simulink model "DCHR_Dispatch_Stateflow_v28"  (R2026a)
settings: Solver=FixedStepDiscrete  StopTime=dchr_stop_v28  FixedStep=dchr_dt_v28
model workspace (MAT data in the model file):
  dchr_E0_v28 = 0
  dchr_dt_v28 = 1
  dchr_h_v28 = [8 0.45 1.2 8 0.08 0 4 0 0]
  dchr_input_v28 = [0  6  35  70  5; 1  0  35  70  6; 2  0  35  70  10]
  dchr_p_v28 = [1 10 3 4 0.9 0.8 0.01 2]
  dchr_stop_v28 = 2
settings Model: Creator=Lysda  LastModifiedBy=Lysda

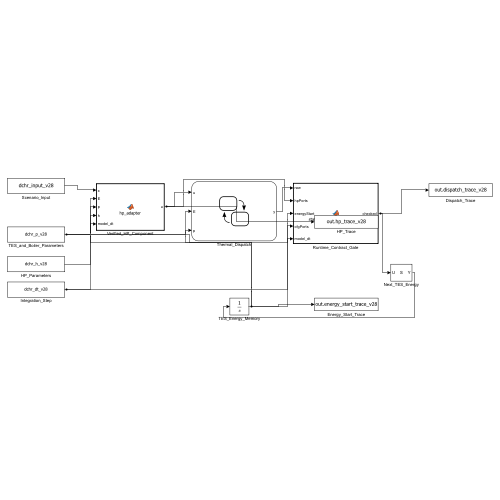
[thumbnail: Simulink's stored preview of the top-level diagram]
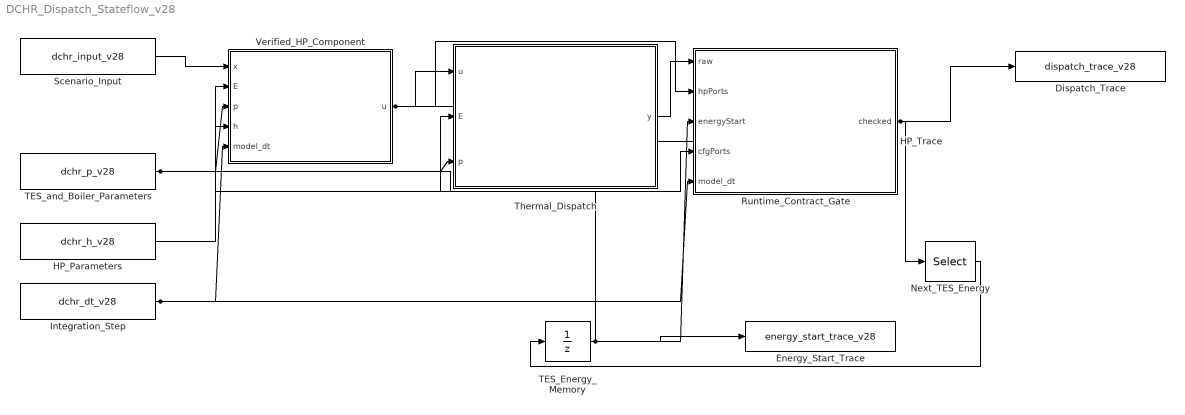
== system DCHR_Dispatch_Stateflow_v28 ==
  Dispatch_Trace : ToWorkspace  VariableName=dispatch_trace_v28  SaveFormat=Timeseries  SampleTime=-1
  Energy_Start_Trace : ToWorkspace  VariableName=energy_start_trace_v28  SaveFormat=Timeseries  SampleTime=-1
  HP_Parameters : Constant  Value=dchr_h_v28
  HP_Trace : ToWorkspace  VariableName=hp_trace_v28  SaveFormat=Timeseries  SampleTime=-1
  Integration_Step : Constant  Value=dchr_dt_v28
  Next_TES_Energy : Selector  InputPortWidth=13  IndexOptions=Index vector (dialog)  Indices=8  OutputSizes=1
  Runtime_Contract_Gate : MATLAB Function  TreatAsAtomicUnit=on
  Scenario_Input : FromWorkspace  VariableName=dchr_input_v28  SampleTime=dchr_dt_v28  Interpolate=off  OutputAfterFinalValue=Holding final value
  TES_Energy_Memory : UnitDelay  InitialCondition=dchr_E0_v28  SampleTime=dchr_dt_v28
  TES_and_Boiler_Parameters : Constant  Value=dchr_p_v28
  Thermal_Dispatch : Stateflow chart  TreatAsAtomicUnit=on
  Verified_HP_Component : MATLAB Function  TreatAsAtomicUnit=on
  wires:
  Scenario_Input/1 -> Verified_HP_Component/1(x)
  TES_Energy_Memory/1 -> Verified_HP_Component/2(E), Thermal_Dispatch/2(E), Runtime_Contract_Gate/3(energyStart), Energy_Start_Trace/1
  TES_and_Boiler_Parameters/1 -> Verified_HP_Component/3(p), Thermal_Dispatch/3(p), Runtime_Contract_Gate/4(cfgPorts)
  HP_Parameters/1 -> Verified_HP_Component/4(h)
  Verified_HP_Component/1(u) -> Thermal_Dispatch/1(u), Runtime_Contract_Gate/2(hpPorts), HP_Trace/1
  Integration_Step/1 -> Verified_HP_Component/5(model_dt), Runtime_Contract_Gate/5(model_dt)
  Thermal_Dispatch/1(y) -> Runtime_Contract_Gate/1(raw)
  Runtime_Contract_Gate/1(checked) -> Next_TES_Energy/1, Dispatch_Trace/1
  Next_TES_Energy/1 -> TES_Energy_Memory/1

== matlab function DCHR_Dispatch_Stateflow_v28/Runtime_Contract_Gate ==
  data: raw input; checked output; hpPorts input; energyStart input; cfgPorts input; model_dt input
function checked = stateflow_contract_gate_v28(raw,hpPorts,energyStart,cfgPorts,model_dt)
%#codegen
% Executed after the operational chart, before accepted trace/TES feedback.
% Powers MW; energies MWh; dt h. Exponential passive retention, LOSS-FIRST split.
% Constant ambient/property lumped assumption; active-flow integration is approximate.
dt=cfgPorts(1); cap=cfgPorts(2); etaC=cfgPorts(5); etaD=cfgPorts(6);
assert(isfinite(model_dt) && model_dt>0 && dt==model_dt, ...
    'Physical interval must equal the model sample time.');
assert(cfgPorts(7)>=0 && isfinite(cfgPorts(7)*dt), 'Invalid continuous loss-rate product.');
assert(all(isfinite(raw)) && all(isfinite(cfgPorts)), ...
    'Accepted dispatch and parameters must be finite.');
assert(all(isfinite(hpPorts([1 2 3 4 5 7 8]))), ...
    'HP ports except off-state COP must be finite.');
% Scale tolerance with total interval energy, never with a reported residual.
scale=max(1,abs(energyStart)+(abs(hpPorts(2))+abs(cfgPorts(8)))*dt+abs(cap));
tol=1e-10*scale;
powerTol=tol/max(dt,eps);
assert(isfinite(scale) && isfinite(tol) && isfinite(powerTol), 'Overflow in contract tolerance.');
assert(energyStart>=0 && energyStart<=cap && cap>=0, 'TES start outside capacity.');
assert(all(raw([2:6 12])>=-powerTol) && all(raw(7:11)>=-tol) && ...
    all(hpPorts([1 2 3 4 5 7 8])>=0), ...
    'Negative dispatch/HP port.');
assert(raw(1)==floor(raw(1)) && raw(1)>=0 && raw(1)<=5, 'Undefined mode.');
assert(raw(3)<=cfgPorts(3)+powerTol && raw(4)<=cfgPorts(4)+powerTol && ...
    raw(5)<=cfgPorts(8)+powerTol, 'TES/backup power limit exceeded.');
assert(raw(7)>=-tol && raw(7)<=cap+tol && raw(8)>=-tol && raw(8)<=cap+tol, ...
    'TES state outside capacity.');
assert(raw(3)*raw(4)==0, 'Simultaneous TES charge and discharge.');
assert(abs(hpPorts(2)-hpPorts(3)-hpPorts(4))*dt<=tol, 'HP first-law failure.');
assert(abs(hpPorts(2)-raw(2)-raw(3))*dt<=tol, 'Unallocated HP condenser heat.');
assert(abs(hpPorts(1)-raw(2)-raw(4)-raw(5)-raw(6))*dt<=tol, 'Demand closure failure.');
assert(abs(raw(12)-raw(2)-raw(4)-raw(5))*dt<=tol, 'Useful heat mismatch.');
assert(abs(raw(7)-energyStart*exp(-cfgPorts(7)*dt))<=tol, 'Standing-retention mismatch.');
assert(abs(raw(9)-(energyStart-raw(7)))<=tol && ...
    abs(raw(10)-(1-etaC)*raw(3)*dt)<=tol && ...
    abs(raw(11)-(1/etaD-1)*raw(4)*dt)<=tol, 'TES loss reporting mismatch.');
tesResidual=energyStart+(raw(3)-raw(4))*dt-raw(8)-sum(raw(9:11));
assert(abs(tesResidual)<=tol, 'TES first-law failure.');
systemResidual=(hpPorts(4)+hpPorts(3)+raw(5))*dt+energyStart ...
    -raw(12)*dt-raw(8)-sum(raw(9:11));
assert(abs(systemResidual)<=tol && abs(raw(13)-systemResidual)<=tol, ...
    'System first-law failure or false residual.');
expected=0;
if raw(6)>0, expected=5;
elseif raw(5)>0, expected=4;
elseif raw(4)>0, expected=3;
elseif raw(3)>0, expected=2;
elseif raw(2)>0, expected=1;
end
assert(raw(1)==expected, 'Active state does not match delivered flows.');
if hpPorts(2)>0
    assert(isfinite(hpPorts(6)) && hpPorts(6)>1 && hpPorts(7)==1, 'Invalid operating COP/availability.');
    assert(abs(hpPorts(3)*hpPorts(6)-hpPorts(2))*dt<=tol, 'COP port inconsistency.');
else
    assert(isnan(hpPorts(6)) && hpPorts(7)==0, 'Off HP must have undefined COP.');
end
checked=raw;
end

== matlab function DCHR_Dispatch_Stateflow_v28/Verified_HP_Component ==
  data: x input; u output; E input; p input; h input; model_dt input
function u=hp_adapter(x,E,p,h,model_dt)
%#codegen
coder.extrinsic('dchr_stateflow_hp_v28');
u=zeros(8,1);
u=dchr_stateflow_hp_v28(x,E,p,h,model_dt);
end

== stateflow chart DCHR_Dispatch_Stateflow_v28/Thermal_Dispatch ==
  settings: updateMethod=DISCRETE  sampleTime=dchr_dt_v28  description=v28 exponential passive TES retention; loss-first split. Six-state finite TES/HP/boiler dispatch. Normal-mode host HP component; state actions drive all delivery ports.
  state IDLE
    en,du:
    y=stateflow_allocate_v28(0,u,E,p);
  state HEAT_RECOVERY
    en,du:
    y=stateflow_allocate_v28(1,u,E,p);
  state STORAGE_CHARGE
    en,du:
    y=stateflow_allocate_v28(2,u,E,p);
  state STORAGE_DISCHARGE
    en,du:
    y=stateflow_allocate_v28(3,u,E,p);
  state BACKUP
    en,du:
    y=stateflow_allocate_v28(4,u,E,p);
  state UNMET_DEMAND
    en,du:
    y=stateflow_allocate_v28(5,u,E,p);
  (junction 22) -> STORAGE_CHARGE [order 3] : [stateflow_choose_mode_v28(u,E,p)==2]
  (junction 22) -> HEAT_RECOVERY [order 2] : [stateflow_choose_mode_v28(u,E,p)==1]
  (default) -> (junction 22)
  (junction 22) -> IDLE [order 1] : [stateflow_choose_mode_v28(u,E,p)==0]
  (junction 22) -> UNMET_DEMAND [order 6] : [stateflow_choose_mode_v28(u,E,p)==5]
  (junction 22) -> STORAGE_DISCHARGE [order 4] : [stateflow_choose_mode_v28(u,E,p)==3]
  (junction 22) -> BACKUP [order 5] : [stateflow_choose_mode_v28(u,E,p)==4]
  STORAGE_CHARGE -> STORAGE_DISCHARGE [order 3] : [stateflow_choose_mode_v28(u,E,p)==3]
  HEAT_RECOVERY -> STORAGE_DISCHARGE [order 3] : [stateflow_choose_mode_v28(u,E,p)==3]
  STORAGE_CHARGE -> BACKUP [order 4] : [stateflow_choose_mode_v28(u,E,p)==4]
  STORAGE_DISCHARGE -> IDLE [order 1] : [stateflow_choose_mode_v28(u,E,p)==0]
  UNMET_DEMAND -> IDLE [order 1] : [stateflow_choose_mode_v28(u,E,p)==0]
  STORAGE_CHARGE -> IDLE [order 1] : [stateflow_choose_mode_v28(u,E,p)==0]
  BACKUP -> IDLE [order 1] : [stateflow_choose_mode_v28(u,E,p)==0]
  HEAT_RECOVERY -> IDLE [order 1] : [stateflow_choose_mode_v28(u,E,p)==0]
  STORAGE_DISCHARGE -> HEAT_RECOVERY [order 2] : [stateflow_choose_mode_v28(u,E,p)==1]
  STORAGE_DISCHARGE -> STORAGE_CHARGE [order 3] : [stateflow_choose_mode_v28(u,E,p)==2]
  BACKUP -> HEAT_RECOVERY [order 2] : [stateflow_choose_mode_v28(u,E,p)==1]
  IDLE -> HEAT_RECOVERY [order 1] : [stateflow_choose_mode_v28(u,E,p)==1]
  IDLE -> STORAGE_CHARGE [order 2] : [stateflow_choose_mode_v28(u,E,p)==2]
  UNMET_DEMAND -> HEAT_RECOVERY [order 2] : [stateflow_choose_mode_v28(u,E,p)==1]
  STORAGE_CHARGE -> HEAT_RECOVERY [order 2] : [stateflow_choose_mode_v28(u,E,p)==1]
  BACKUP -> STORAGE_CHARGE [order 3] : [stateflow_choose_mode_v28(u,E,p)==2]
  UNMET_DEMAND -> STORAGE_CHARGE [order 3] : [stateflow_choose_mode_v28(u,E,p)==2]
  HEAT_RECOVERY -> STORAGE_CHARGE [order 2] : [stateflow_choose_mode_v28(u,E,p)==2]
  IDLE -> STORAGE_DISCHARGE [order 3] : [stateflow_choose_mode_v28(u,E,p)==3]
  HEAT_RECOVERY -> BACKUP [order 4] : [stateflow_choose_mode_v28(u,E,p)==4]
  STORAGE_CHARGE -> UNMET_DEMAND [order 5] : [stateflow_choose_mode_v28(u,E,p)==5]
  IDLE -> BACKUP [order 4] : [stateflow_choose_mode_v28(u,E,p)==4]
  IDLE -> UNMET_DEMAND [order 5] : [stateflow_choose_mode_v28(u,E,p)==5]
  HEAT_RECOVERY -> UNMET_DEMAND [order 5] : [stateflow_choose_mode_v28(u,E,p)==5]
  UNMET_DEMAND -> STORAGE_DISCHARGE [order 4] : [stateflow_choose_mode_v28(u,E,p)==3]
  BACKUP -> STORAGE_DISCHARGE [order 4] : [stateflow_choose_mode_v28(u,E,p)==3]
  STORAGE_DISCHARGE -> BACKUP [order 4] : [stateflow_choose_mode_v28(u,E,p)==4]
  STORAGE_DISCHARGE -> UNMET_DEMAND [order 5] : [stateflow_choose_mode_v28(u,E,p)==5]
  UNMET_DEMAND -> BACKUP [order 5] : [stateflow_choose_mode_v28(u,E,p)==4]
  BACKUP -> UNMET_DEMAND [order 5] : [stateflow_choose_mode_v28(u,E,p)==5]
  data: hpPorts function_input; energyStart function_input; cfgPorts function_input; mode function_output; mode function_input; hpPorts function_input; energyStart function_input; cfgPorts function_input; y function_output; u input double size=[8 1]; E input double size=1; p input double size=[1 8]; y output double size=[13 1]
  function mode = stateflow_choose_mode_v28(hpPorts,energyStart,cfgPorts):
    | function mode = stateflow_choose_mode_v28(hpPorts,energyStart,cfgPorts)
    | %#codegen
    | % Highest service condition; BACKUP/UNMET can include HP and TES discharge.
    | % hpPorts = [demand, HP heat, electricity, source used, request, COP, available, unused]
    | % cfgPorts = [dt_h, capacity, charge limit, discharge limit, etaC, etaD, continuous lambda/h, boiler]
    | after=energyStart*exp(-cfgPorts(7)*cfgPorts(1));
    | direct=min(hpPorts(1),hpPorts(2));
    | discharge=min([max(0,hpPorts(1)-direct),cfgPorts(4),after*cfgPorts(6)/cfgPorts(1)]);
    | remaining=max(0,hpPorts(1)-direct-discharge);
    | if remaining>cfgPorts(8)
    |     mode=5;
    | elseif remaining>0
    |     mode=4;
    | elseif discharge>0
    |     mode=3;
    | elseif hpPorts(2)>direct
    |     mode=2;
    | elseif direct>0
    |     mode=1;
    | else
    |     mode=0;
    | end
    | end
  function y = stateflow_allocate_v28(mode,hpPorts,energyStart,cfgPorts):
    | function y = stateflow_allocate_v28(mode,hpPorts,energyStart,cfgPorts)
    | %#codegen
    | % Called by the active Stateflow state's entry and during actions.
    | % States determine which TES/backup/unmet ports may operate.
    | dt=cfgPorts(1); after=energyStart*exp(-cfgPorts(7)*dt);
    | direct=0; charge=0; discharge=0; gas=0; unmet=0;
    | if mode>=1
    |     direct=min(hpPorts(1),hpPorts(2));
    | end
    | if mode==2
    |     charge=min([max(0,hpPorts(2)-direct),cfgPorts(3),(cfgPorts(2)-after)/dt/cfgPorts(5)]);
    | end
    | if mode>=3
    |     discharge=min([max(0,hpPorts(1)-direct),cfgPorts(4),after*cfgPorts(6)/dt]);
    | end
    | if mode>=4
    |     gas=min(cfgPorts(8),max(0,hpPorts(1)-direct-discharge));
    | end
    | if mode==5
    |     unmet=max(0,hpPorts(1)-direct-discharge-gas);
    | end
    | next=min(cfgPorts(2),max(0,after+cfgPorts(5)*charge*dt-discharge*dt/cfgPorts(6)));
    | standing=-energyStart*expm1(-cfgPorts(7)*dt);
    | chargeLoss=(1-cfgPorts(5))*charge*dt;
    | dischargeLoss=discharge*dt/cfgPorts(6)-discharge*dt;
    | supplied=direct+discharge+gas;
    | residual=(hpPorts(4)+hpPorts(3)+gas)*dt+energyStart-supplied*dt-next-standing-chargeLoss-dischargeLoss;
    | y=[mode;direct;charge;discharge;gas;unmet;after;next;standing;chargeLoss;dischargeLoss;supplied;residual];
    | end
